simulink model "ecu_rail"  (R2026a)
settings: Solver=FixedStepDiscrete  StopTime=10  FixedStep=0.001  SampleTimeConstraint=STIndependent
Description:
  | Rail-pressure PI. Source of truth for firmware/gen/ecu_rail.
settings Model: Creator=jj1001000  LastModifiedBy=jj1001000
settings OptimizationCC: DefaultUnderspecifiedDataType=single
settings DebuggingCC: ParameterPrecisionLossMsg=none
settings HardwareCC: ProdLargestAtomicInteger=Long  ProdLargestAtomicFloat=Double  ProdHWDeviceType=ARM Compatible->ARM Cortex-M
settings RTWCC: SystemTargetFile=ert.tlc  GenCodeOnly=on  Description=Embedded Coder
settings ERTTargetCC: UtilityFuncGeneration=Shared location  IncludeMdlTerminateFcn=off  CodeInterfacePackaging=Reusable function  SupportNonFinite=off

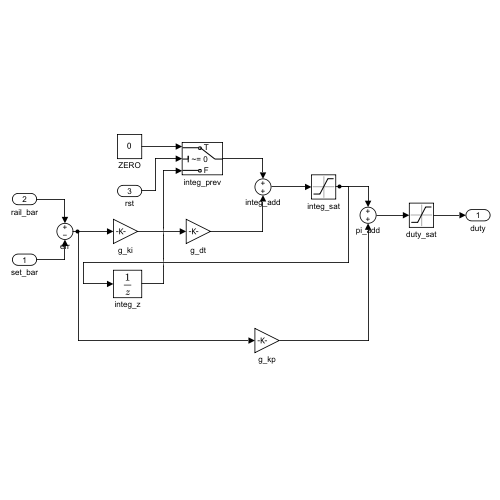
[thumbnail: Simulink's stored preview of the top-level diagram]
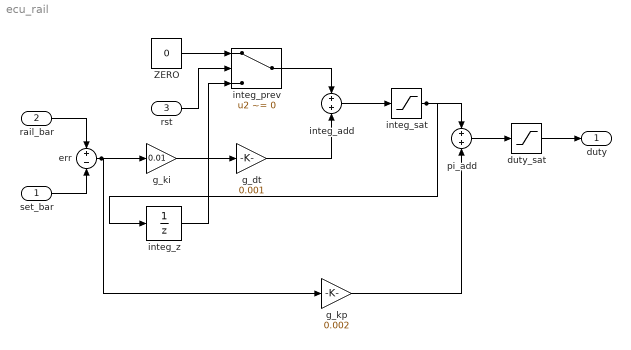
== system ecu_rail ==
  set_bar : Inport  OutDataTypeStr=single
  rail_bar : Inport  Port=2  OutDataTypeStr=single
  rst : Inport  Port=3  OutDataTypeStr=uint8
  ZERO : Constant  Value=0  OutDataTypeStr=single
  duty_sat : Saturate  UpperLimit=1  LowerLimit=0
  err : Sum  Inputs=+-
  g_dt : Gain  Gain=0.001
  g_ki : Gain  Gain=0.01
  g_kp : Gain  Gain=0.002
  integ_add : Sum
  integ_prev : Switch  Criteria=u2 ~= 0  SaturateOnIntegerOverflow=off  InputSameDT=off
  integ_sat : Saturate  UpperLimit=1  LowerLimit=0
  integ_z : UnitDelay  SampleTime=-1
  pi_add : Sum
  duty : Outport  OutDataTypeStr=single
  wires:
  set_bar/1 -> err/2
  rst/1 -> integ_prev/2
  rail_bar/1 -> err/1
  err/1 -> g_kp/1, g_ki/1
  integ_z/1 -> integ_prev/3
  ZERO/1 -> integ_prev/1
  g_ki/1 -> g_dt/1
  integ_prev/1 -> integ_add/1
  integ_add/1 -> integ_sat/1
  g_dt/1 -> integ_add/2
  g_kp/1 -> pi_add/2
  integ_sat/1 -> integ_z/1, pi_add/1
  pi_add/1 -> duty_sat/1
  duty_sat/1 -> duty/1
